simulink model "EINT_system_simulation"  (R2026b)
settings: Solver=FixedStepAuto  StopTime=10  FixedStep=Ts
values from neighbouring files (symbols this model uses):
  Ts = 0.05    [generate_commande_preview.m]    (also in random_init.m)
settings Model: Creator=Max  LastModifiedBy=ctamboise

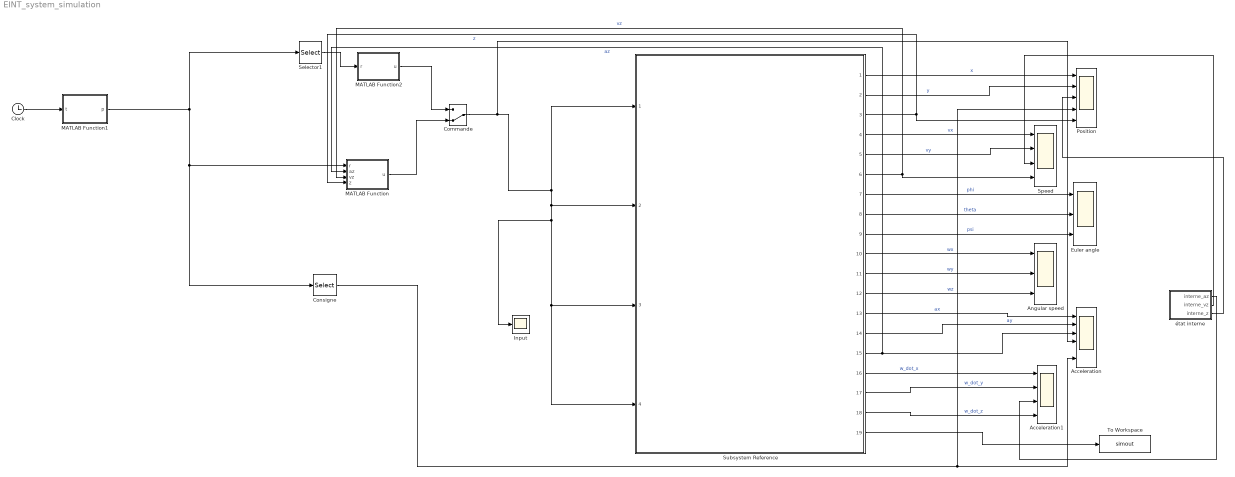
== system EINT_system_simulation ==
  Acceleration : Scope  NumInputPorts=6
      settings: ActiveDisplayYMinimum=-16.009651030181232  ActiveDisplayYMaximum=12.80304299762131
  Acceleration1 : Scope  NumInputPorts=4
      settings: ActiveDisplayYMinimum=-40.918121722117149  ActiveDisplayYMaximum=44.001627281329164  DataLoggingVariableName=ScopeData2
  Angular speed : Scope  NumInputPorts=3
      settings: ActiveDisplayYMinimum=-1  ActiveDisplayYMaximum=1  DataLoggingVariableName=ScopeData3
  Clock : Clock
  Commande : ManualSwitch  CurrentSetting=0
  Consigne : Selector  InputPortWidth=20  IndexOptions=Index vector (dialog)  Indices=1  OutputSizes=1  RuntimeRangeChecks=off
  Euler angle : Scope  NumInputPorts=3
      settings: ActiveDisplayYMinimum=-1695.66598  ActiveDisplayYMaximum=1344.64163  DataLoggingVariableName=ScopeData4
  Input : Scope
      settings: ActiveDisplayYMinimum=-1.25  ActiveDisplayYMaximum=1.25  DataLoggingVariableName=ScopeData5
  MATLAB Function : MATLAB Function  TreatAsAtomicUnit=on
  MATLAB Function1 : MATLAB Function  TreatAsAtomicUnit=on
  MATLAB Function2 : MATLAB Function  TreatAsAtomicUnit=on
  Position : Scope  NumInputPorts=5
      settings: ActiveDisplayYMinimum=-0.30617427592313462  ActiveDisplayYMaximum=0.646531888678924  DataLoggingVariableName=ScopeData6
  Selector1 : Selector  InputPortWidth=20  IndexOptions=Index vector (dialog)  Indices=1  OutputSizes=1  RuntimeRangeChecks=off
  Speed : Scope  NumInputPorts=4
      settings: ActiveDisplayYMinimum=-2.0291599170695513  ActiveDisplayYMaximum=0.93228871088825449
  Subsystem Reference : Subsystem  ReferencedSubsystem=UAV_model
  To Workspace : ToWorkspace  VariableName=simout  SaveFormat=Structure With Time  SampleTime=Ts
  état interne : MATLAB Function  TreatAsAtomicUnit=on
  wires:
  Subsystem Reference/18 -> Acceleration1/4  "w_dot_z"
  Subsystem Reference/12 -> Angular speed/3  "wz"
  Subsystem Reference/17 -> Acceleration1/2  "w_dot_y"
  Subsystem Reference/9 -> Euler angle/3  "psi"
  Subsystem Reference/8 -> Euler angle/2  "theta"
  Subsystem Reference/14 -> Acceleration/2  "ay"
  Subsystem Reference/10 -> Angular speed/1  "wx"
  Subsystem Reference/2 -> Position/2  "y"
  Subsystem Reference/13 -> Acceleration/1  "ax"
  Subsystem Reference/15 -> MATLAB Function/2(az), Acceleration/3  "az"
  Subsystem Reference/16 -> Acceleration1/1  "w_dot_x"
  Subsystem Reference/7 -> Euler angle/1  "phi"
  Subsystem Reference/19 -> To Workspace/1
  Subsystem Reference/1 -> Position/1  "x"
  Subsystem Reference/6 -> MATLAB Function/3(vz), Speed/4  "vz"
  Subsystem Reference/4 -> Speed/1  "vx"
  Subsystem Reference/3 -> MATLAB Function/4(z), Position/5  "z"
  Subsystem Reference/5 -> Speed/2  "vy"
  Subsystem Reference/11 -> Angular speed/2  "wy"
  Clock/1 -> MATLAB Function1/1(t)
  Consigne/1 -> Position/4, Acceleration/6
  Selector1/1 -> MATLAB Function2/1(r)
  MATLAB Function2/1(u) -> Commande/1
  Commande/1 -> Acceleration/4, Subsystem Reference/4, Subsystem Reference/3, Input/1, Subsystem Reference/2, Subsystem Reference/1
  MATLAB Function1/1(p) -> Consigne/1, MATLAB Function/1(r), Selector1/1
  MATLAB Function/1(u) -> Commande/2
  état interne/3(interne_z) -> Position/3
  état interne/1(interne_az) -> Acceleration1/3
  état interne/2(interne_vz) -> Speed/3

== matlab function EINT_system_simulation/MATLAB Function ==
  data: r input; u output; az input; vz input; z input
function u = mpc_controller_block(r,az, vz, z)
%#codegen
persistent controller

coder.extrinsic('evalin', 'step');

u = 0.0;

if isempty(controller)
    controller = evalin('base', 'mpc_system');
end

u = step(controller, r, az, vz, z);
end

== matlab function EINT_system_simulation/MATLAB Function1 ==
  data: t input; p output
function p = space_command(t)
    coder.extrinsic('commande_space_step');
    p = zeros(1,3);
    p = commande_space_step(t);
end

== matlab function EINT_system_simulation/MATLAB Function2 ==
  data: r input; u output
function u = linear_controller_block(r)
%#codegen
persistent controller

% Déclarer les fonctions MATLAB non générables en C comme extrinsèques
coder.extrinsic('evalin', 'step');

% Définir le type et la taille de la sortie Simulink
u = 0.0;

% Récupérer l'instance mpc_system du Workspace MATLAB au 1er pas de temps
if isempty(controller)
    controller = evalin('base', 'linear_system');
end

% Appeler la méthode step() à chaque pas de temps de simulation
u = step(controller, r);
end

== matlab function EINT_system_simulation/état interne ==
  data: interne_az output; interne_vz output; interne_z output
function [interne_az, interne_vz, interne_z] = mpc_state_block()
%#codegen

% Déclaration de la fonction externe
coder.extrinsic('mpc_internal_state');

% 1. Initialisation des types et tailles de sortie
az = 0.0;
vz = 0.0;
z  = 0.0;

% 2. PRÉ-ALLOCATION de 'res' (Obligatoire pour coder.extrinsic)
% Cela indique au compilateur Simulink que 'res' sera un tableau de doubles 3x1
res = zeros(3, 1);

% 3. Appel extrinsèque de la fonction MATLAB (qui appelle Python)
if nargin > 0
    res = mpc_internal_state(u);
else
    res = mpc_internal_state();
end

% 4. Extraction des composantes
interne_az = res(1);
interne_vz = res(2);
interne_z  = res(3);
end
